simulink model "SIM_SFC_TEMPLATE"  (R2024b)
settings: Solver=FixedStepAuto  StartTime=0.0  StopTime=TSim  FixedStep=Ts  RelTol=1e-3
InitFcn:
  | load('LoadParameters_SFC2K.mat')
settings Model: Creator=rmrane  LastModifiedBy=vreyesdreke
settings OptimizationCC: DefaultParameterBehavior=Inlined  EnhancedBackFolding=on  PassReuseOutputArgsAs=Individual arguments  ZeroExternalMemoryAtStartup=off  ZeroInternalMemoryAtStartup=off  OptimizeBlockOrder=speed  DifferentSizesBufferReuse=on  OptimizationCustomize=off  EfficientTunableParamExpr=on
settings DebuggingCC: ParameterTunabilityLossMsg=error
settings SFSimCC: MATLABDynamicMemAlloc=off
settings RTWCC: Description=Embedded Coder  SystemTargetFile=ert.tlc  TemplateMakefile=ert_default_tmf
settings CodeAppCC: GenerateComments=off  IgnoreCustomStorageClasses=off  OperatorAnnotations=on  SimulinkDataObjDesc=on  SFDataObjDesc=on  CustomSymbolStrType=$N$R$M  SimulinkBlockComments=off  InternalIdentifier=Classic
settings ERTTargetCC: GenerateSampleERTMain=on  SupportAbsoluteTime=off  SupportNonFinite=off  SupportComplex=off  ERTCustomFileTemplate=example_file_process.tlc  ConvertIfToSwitch=off  SuppressUnreachableDefaultCases=off  EnableSignedLeftShifts=off  EnableSignedRightShifts=off  DynamicArrayContainerType=coder::array

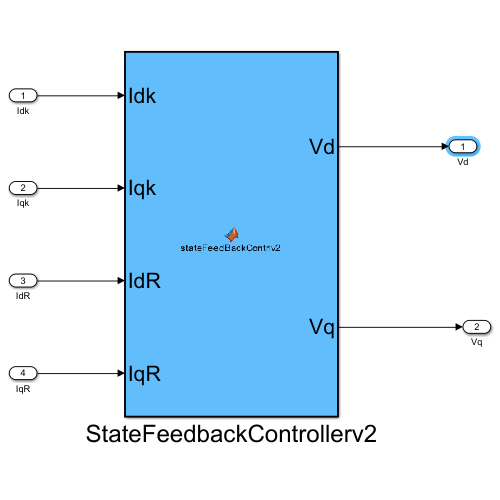
[thumbnail: Simulink's stored preview of the top-level diagram]
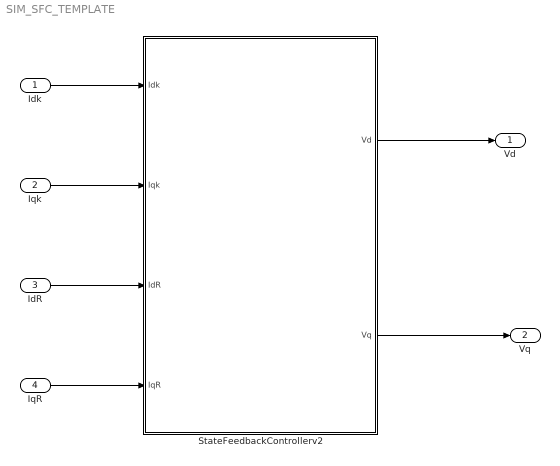
== system SIM_SFC_TEMPLATE ==
  Idk : Inport
  Iqk : Inport  Port=2
  IdR : Inport  Port=3
  IqR : Inport  Port=4
  StateFeedbackControllerv2 : MATLAB Function  TreatAsAtomicUnit=on
  Vd : Outport
  Vq : Outport  Port=2
  wires:
  Idk/1 -> StateFeedbackControllerv2/1(Idk)
  Iqk/1 -> StateFeedbackControllerv2/2(Iqk)
  IdR/1 -> StateFeedbackControllerv2/3(IdR)
  IqR/1 -> StateFeedbackControllerv2/4(IqR)
  StateFeedbackControllerv2/1(Vd) -> Vd/1
  StateFeedbackControllerv2/2(Vq) -> Vq/1

== matlab function SIM_SFC_TEMPLATE/StateFeedbackControllerv2 ==
  settings: updateMethod=DISCRETE  sampleTime=Ts
  data: Idk input size=1; Vd output size=1; Vq output size=1; Iqk input size=1; IdR input size=1; IqR input size=1
function [Vd,Vq] = stateFeedBackContrlv2(Idk,Iqk,IdR,IqR)
% stateFeedBackContrl(Idk,Iqk,IdP,IqP,IdR,IqR,uk0)
% MATLAB fcn to implement the state-feedback controller in RSCAD. This
% state feedback control law is tailored for OCC of MMCs. 
% ------------------------------
% Pseudo-code
% xk = [Idk-IdP,Iqk-IqP,Idk,Iqk]';
% rk = [0, 0, IdR, IqR]';
% ek = xk-rk;
% uk = (K*ek)+uk0;
% ------------------------------
% Load precomputed matrices
S = coder.load('LoadParameters_SFC2K.mat','-mat','-regexp','K','Kuss');
% ------------------------------    
% Computation
uk =  (S.K*(-[IdR; IqR]+[Idk;Iqk]))+S.Kuss*[IdR; IqR];
Vd = uk(1);  
Vq = uk(2);
